simulink model "ps_model"  (R2025b)
settings: Solver=ode23tb  StartTime=0.0  StopTime=simlength  FixedStep=tc  MaxStep=tc
values from neighbouring files (symbols this model uses):
  omega_grid_emulator_nom = w_grid    (= 314.159265359)    [grid_emulator.m]
  omega_grid_nom = w_grid    (= 314.159265359)    [grid_emulator.m]
  ugrid_factor = 1    [grid_emulator.m]
  V_phase_normalization_factor = Vgrid_phase_normalization_factor    [grid_emulator.m]
  Vdc_base = 720    [grid_emulator.m]
  vn_eta_pu = 0    [grid_emulator.m]
  vn_xi_pu = 0    [grid_emulator.m]
  vp_xi_pu = 1    [grid_emulator.m]
undefined symbols (not defined in the file or in its folder): CFi, fnom, fPWM_INV, i_nom, ki_i, ki_u, kp_i, kp_u, Ld2_trafo_out, magnitude, n10, number_of_cells, omega_nom, Q, q1Kalman, q2Kalman, q3Kalman, R_RLload, Rd2_trafo_out, rKalman, tc, time_load_step, ts_afe, ts_inv, tsample, u_nom, Vdc_nom
libraries: fl_lib x120, nesl_utility x67, ee_lib x7, cstblocks x4, moving_average_filter x4, single_phase_transformer_lib x3, lithium_ion_cell_lib x1, simulink x1, threephase_inductor_lib x1
(part 1 of 4)
settings Model: SimulationMode=accelerator  Creator=dbagn  LastModifiedBy=dbagn
settings SolverCC: NumberNewtonIterations=3.0  ZeroCrossControl=DisableAll  AlgebraicLoopSolver=TrustRegion  SolverResetMethod=Robust
settings DataIOCC: SaveOutput=off  SignalLogging=off  DSMLogging=off  SaveTime=off  ReturnWorkspaceOutputs=off
settings OptimizationCC: ReuseModelBlockBuffer=off
settings DebuggingCC: UnconnectedInputMsg=warning  UnconnectedOutputMsg=warning  UnconnectedLineMsg=warning
settings ModelReferenceCC: EnableRefExpFcnMdlSchedulingChecks=on
settings SFSimCC: SimUserIncludeDirs=include  SimAnalyzeCustomCode=on
settings SFSimCC: SimCustomHeaderCode=|
  | #include "mavgflt.h"
  | #include "bemf_obsv.h"
  | #include "dqvector_pi.h"
  | #include "dqvector_pi_simulink.h"
  | #include "mavgflt_simulink.h"
  | #include "sv_pwm.h"
  | #include "bemf_obsv_simulink.h"
  | #include "bemf_obsv_load_est.h"
  | #include "bemf_obsv_load_est_simulink.h"
  | #include "sv_pwm_simulink.h"
  | #include "fb_state_machine.h"
  | #include "fb_state_machine_simulink.h"
settings SFSimCC: SimUserSources=|
  | dqvector_pi.c
  | dqvector_pi_simulink.c
  | mavgflt_simulink.c
  | mavgflt.c
  | bemf_obsv_simulink.c
  | bemf_obsv.c
  | bemf_obsv_load_est_simulink.c
  | bemf_obsv_load_est.c
  | sv_pwm.c
  | sv_pwm_simulink.c
  | fb_state_machine.c
  | fb_state_machine_simulink.c
settings RTWCC: GPUComputeCapability=3.5  DLArmComputeVersion=19.05

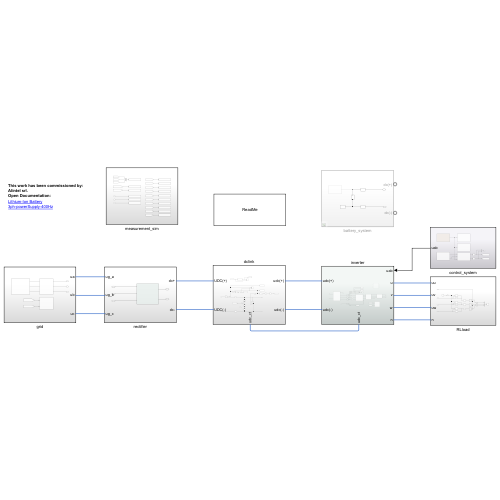
[thumbnail: Simulink's stored preview of the top-level diagram]
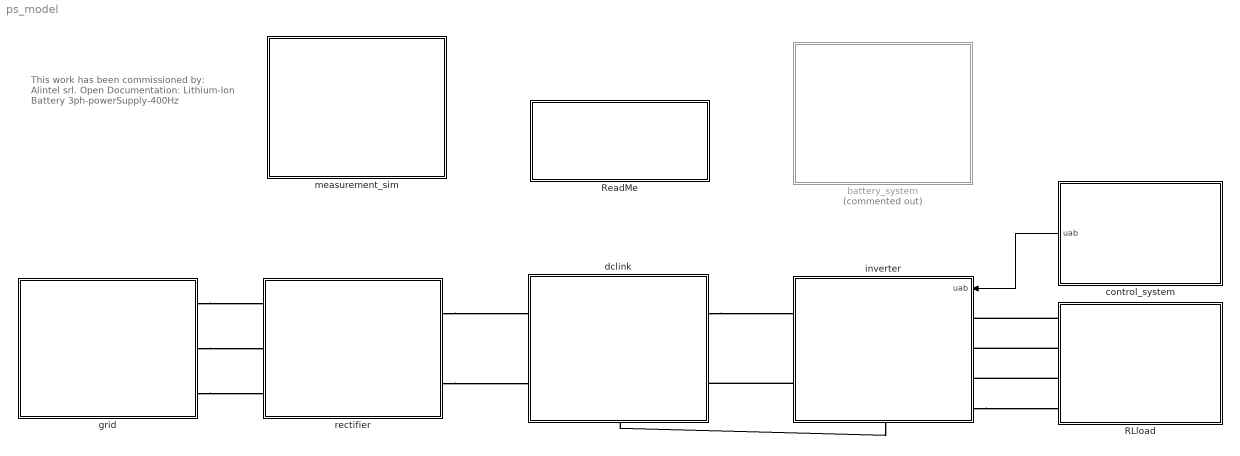
== system ps_model ==
  note: This work has been commissioned by:
      | Alintel srl.
      | Open Documentation:
      | Lithium-Ion Battery
      | 3ph-powerSupply-400Hz
  RLload : Subsystem
  ReadMe : Subsystem
      mask Display: disp('ReadMe')
  battery_system : Subsystem  Commented=on
  control_system : Subsystem
  dclink : Subsystem
      settings: PortSchema="{\"entries\":[{\"content\":{\"sides\":[{\"content\":{\"connectorIds\":[\"LConn1\",\"LConn2\"]},\"type\":\"ConnectorPlacement.EquallySpacedRectSide\",\"uuid\":\"065d3cf8-4b88-4bd8-afed-5c791b4c8227\"},{\"content\":{\"connectorIds\":[\"RConn1\",\"RConn2\"],\"side\":\"RIGHT\"},\"type\":\"ConnectorPlacement.EquallySpacedRectSide\",\"uuid\":\"93da4eee-d833-4749-b194-724bf2a8184c\"},{\"content\":{\"side\":\"TOP\"},\"type\":\"ConnectorPlacement.EquallySpacedRectSide\",\"uuid\":\"7e72ab0b-6fa9-40de-a645-1ec9cfd9e31f\"},{\"content\":{\"connectorIds\":[\"RConn3\"],\"side\":\"BOTTOM\"},\"type\":\"ConnectorPlacement.EquallySpacedRectSide\",\"uuid\":\"310375c4-299b-412a-a0fa-962bdc2b4f11\"}]},\"type\":\"ConnectorPlacement.EquallySpacedConnector\",\"uuid\":\"547429aa-4b93-405e-bc45-7aab171afd7d\"}],\"packageUris\":[\"http://schema.mathworks.com/mf0/Connector/R2020b\"],\"version\":\"1.0\"}"
  grid : Subsystem
  inverter : Subsystem
      settings: PortSchema="{\"entries\":[{\"content\":{\"sides\":[{\"content\":{\"connectorIds\":[\"In1\",\"LConn1\",\"LConn2\",\"LConn3\",\"LConn4\"]},\"type\":\"ConnectorPlacement.EquallySpacedRectSide\",\"uuid\":\"f55c1ca8-6919-4d30-91be-29ab6e5a5b93\"},{\"content\":{\"connectorIds\":[\"RConn1\",\"RConn2\"],\"side\":\"RIGHT\"},\"type\":\"ConnectorPlacement.EquallySpacedRectSide\",\"uuid\":\"500f40ac-770d-4aaa-b814-72c952c48909\"},{\"content\":{\"side\":\"TOP\"},\"type\":\"ConnectorPlacement.EquallySpacedRectSide\",\"uuid\":\"36360c7a-d142-42b5-a71d-dca271faa73f\"},{\"content\":{\"connectorIds\":[\"RConn3\"],\"side\":\"BOTTOM\"},\"type\":\"ConnectorPlacement.EquallySpacedRectSide\",\"uuid\":\"19fec778-0473-49a4-aa84-7932c0a6b289\"}]},\"type\":\"ConnectorPlacement.EquallySpacedConnector\",\"uuid\":\"7d88957d-a3a4-4eee-9ba8-53fe19feea5c\"}],\"packageUris\":[\"http://schema.mathworks.com/mf0/Connector/R2020b\"],\"version\":\"1.0\"}"
  measurement_sim : Subsystem
  rectifier : Subsystem
  wires:
  control_system/1(uab) -> inverter/1(uab)
  connections:
  rectifier/RConn1 -- dclink/LConn1
  rectifier/RConn2 -- dclink/LConn2
  inverter/RConn2 -- dclink/RConn2
  dclink/RConn1 -- inverter/RConn1
  RLload/LConn3 -- inverter/LConn3
  RLload/LConn2 -- inverter/LConn2
  RLload/LConn1 -- inverter/LConn1
  grid/RConn1 -- rectifier/LConn1
  grid/RConn2 -- rectifier/LConn2
  grid/RConn3 -- rectifier/LConn3
  inverter/RConn3 -- dclink/RConn3
  inverter/LConn4 -- RLload/LConn4

== system ps_model/RLload ==
  Bus Creator1 : BusCreator  Inputs=3
  Current Sensor : fl_lib/Electrical/Electrical Sensors/Current Sensor
  Current Sensor1 : fl_lib/Electrical/Electrical Sensors/Current Sensor
  Current Sensor2 : fl_lib/Electrical/Electrical Sensors/Current Sensor
  Inductor : ee_lib/Passive/Inductor  l=L_RLload H  enable_L_tol=0  L_tol=20  tol_distribution=1  nSigma=4  r=0 Ohm  g=1e-9 1/Ohm  enable_operating_limits=0  operating_limit_action=2  max_working_current=1 A  power_rating=1 W  i_L_specify=off  i_L_priority=High  i_L=0 A  i_L_nominal_specify=off  i_L_nominal_value=1  i_L_nominal_unit=A
  Inductor1 : ee_lib/Passive/Inductor  l=L_RLload H  enable_L_tol=0  L_tol=20  tol_distribution=1  nSigma=4  r=0 Ohm  g=1e-9 1/Ohm  enable_operating_limits=0  operating_limit_action=2  max_working_current=1 A  power_rating=1 W  i_L_specify=off  i_L_priority=High  i_L=0 A  i_L_nominal_specify=off  i_L_nominal_value=1  i_L_nominal_unit=A
  Inductor2 : ee_lib/Passive/Inductor  l=L_RLload H  enable_L_tol=0  L_tol=20  tol_distribution=1  nSigma=4  r=0 Ohm  g=1e-9 1/Ohm  enable_operating_limits=0  operating_limit_action=2  max_working_current=1 A  power_rating=1 W  i_L_specify=off  i_L_priority=High  i_L=0 A  i_L_nominal_specify=off  i_L_nominal_value=1  i_L_nominal_unit=A
  PS-Simulink Converter1 : nesl_utility/PS-Simulink Converter  PhysicalDomain=network_engine_domain  SubClassName=ps_output  LeftPortType=input  RightPortType=output  PseudoPeriodic=off  Frequencies=[]  VectorFormat=1-D array  Unit=A  AffineConversion=off
  PS-Simulink Converter2 : nesl_utility/PS-Simulink Converter  PhysicalDomain=network_engine_domain  SubClassName=ps_output  LeftPortType=input  RightPortType=output  PseudoPeriodic=off  Frequencies=[]  VectorFormat=1-D array  Unit=A  AffineConversion=off
  PS-Simulink Converter3 : nesl_utility/PS-Simulink Converter  PhysicalDomain=network_engine_domain  SubClassName=ps_output  LeftPortType=input  RightPortType=output  PseudoPeriodic=off  Frequencies=[]  VectorFormat=1-D array  Unit=A  AffineConversion=off
  Resistor : fl_lib/Electrical/Electrical Elements/Resistor  R=R_RLload Ohm  i_specify=off  i_priority=None  i=0 A  i_nominal_specify=off  i_nominal_value=1  i_nominal_unit=A  v_specify=off  v_priority=None  v=0 V  v_nominal_specify=off  v_nominal_value=1  v_nominal_unit=V
  Resistor1 : fl_lib/Electrical/Electrical Elements/Resistor  R=R_RLload Ohm  i_specify=off  i_priority=None  i=0 A  i_nominal_specify=off  i_nominal_value=1  i_nominal_unit=A  v_specify=off  v_priority=None  v=0 V  v_nominal_specify=off  v_nominal_value=1  v_nominal_unit=V
  Resistor2 : fl_lib/Electrical/Electrical Elements/Resistor  R=R_RLload Ohm  i_specify=off  i_priority=None  i=0 A  i_nominal_specify=off  i_nominal_value=1  i_nominal_unit=A  v_specify=off  v_priority=None  v=0 V  v_nominal_specify=off  v_nominal_value=1  v_nominal_unit=V
  Simulink-PS Converter : nesl_utility/Simulink-PS Converter  PhysicalDomain=network_engine_domain  SubClassName=ps_input  LeftPortType=input  RightPortType=output  PseudoPeriodic=off  Frequencies=[]  NoiseDistribution=none  NoiseParameters=[]  Unit=1  AffineConversion=off  FilteringAndDerivatives=provide  SimscapeFilterOrder=1  InputFilterTimeConstant=0.001  UdotUserProvided=0
  Step : Step  Time=time_load_step  SampleTime=0
  Switch : fl_lib/Electrical/Electrical Elements/Switch  R_closed=0.8 Ohm  G_open=1e-8 1/Ohm  Threshold=0.5  i_specify=off  i_priority=None  i=0 A  i_nominal_specify=off  i_nominal_value=1  i_nominal_unit=A  v_specify=off  v_priority=None  v=0 V  v_nominal_specify=off  v_nominal_value=1  v_nominal_unit=V
  Switch1 : fl_lib/Electrical/Electrical Elements/Switch  R_closed=0.8 Ohm  G_open=1e-8 1/Ohm  Threshold=0.5  i_specify=off  i_priority=None  i=0 A  i_nominal_specify=off  i_nominal_value=1  i_nominal_unit=A  v_specify=off  v_priority=None  v=0 V  v_nominal_specify=off  v_nominal_value=1  v_nominal_unit=V
  Switch2 : fl_lib/Electrical/Electrical Elements/Switch  R_closed=0.8 Ohm  G_open=1e-8 1/Ohm  Threshold=0.5  i_specify=off  i_priority=None  i=0 A  i_nominal_specify=off  i_nominal_value=1  i_nominal_unit=A  v_specify=off  v_priority=None  v=0 V  v_nominal_specify=off  v_nominal_value=1  v_nominal_unit=V
  iuvw_load : Scope
      settings: SampleTime=tc  ActiveDisplayYMinimum=-395.78182  ActiveDisplayYMaximum=375.94765
  uu : PMIOPort  Side=Left
  uv : PMIOPort  Port=2  Side=Left
  uw : PMIOPort  Port=3  Side=Left
  n : PMIOPort  Port=4  Side=Left
  wires:
  PS-Simulink Converter1/1 -> Bus Creator1/1  "iu_load_sim"
  Bus Creator1/1 -> iuvw_load/1
  PS-Simulink Converter3/1 -> Bus Creator1/3  "iw_load_sim"
  PS-Simulink Converter2/1 -> Bus Creator1/2  "iv_load_sim"
  Step/1 -> Simulink-PS Converter/1
  connections:
  uv/RConn1 -- Switch1/RConn2 -- Resistor1/LConn1
  Resistor/LConn1 -- uu/RConn1 -- Switch/RConn2
  uw/RConn1 -- Switch2/RConn2 -- Resistor2/LConn1
  Resistor1/RConn1 -- Switch1/LConn1 -- Inductor1/LConn1
  Switch/LConn1 -- Resistor/RConn1 -- Inductor/LConn1
  Inductor2/LConn1 -- Switch2/LConn1 -- Resistor2/RConn1
  PS-Simulink Converter3/LConn1 -- Current Sensor2/RConn1
  Current Sensor1/RConn1 -- PS-Simulink Converter2/LConn1
  Current Sensor/RConn2 -- Current Sensor2/RConn2 -- Current Sensor1/RConn2 -- n/RConn1
  Current Sensor/RConn1 -- PS-Simulink Converter1/LConn1
  Current Sensor/LConn1 -- Inductor/RConn1
  Inductor2/RConn1 -- Current Sensor2/LConn1
  Inductor1/RConn1 -- Current Sensor1/LConn1
  Switch/RConn1 -- Simulink-PS Converter/RConn1 -- Switch2/RConn1 -- Switch1/RConn1

== system ps_model/ReadMe ==

== system ps_model/battery_system ==
  DC Voltage Source : fl_lib/Electrical/Electrical Sources/DC Voltage Source  v0=Vdc_ref V
  Inductor : fl_lib/Electrical/Electrical Elements/Inductor  l=100e-6 H  r=0.025 Ohm  g=1e-9 1/Ohm  i_specify=off  i_priority=None  i=0 A  i_nominal_specify=off  i_nominal_value=1  i_nominal_unit=A  v_specify=off  v_priority=None  v=0 V  v_nominal_specify=off  v_nominal_value=1  v_nominal_unit=V  i_L_specify=off  i_L_priority=High  i_L=0 A  i_L_nominal_specify=off  i_L_nominal_value=1  i_L_nominal_unit=A
  Inductor1 : fl_lib/Electrical/Electrical Elements/Inductor  l=100e-6 H  r=0.025 Ohm  g=1e-9 1/Ohm  i_specify=off  i_priority=None  i=0 A  i_nominal_specify=off  i_nominal_value=1  i_nominal_unit=A  v_specify=off  v_priority=None  v=0 V  v_nominal_specify=off  v_nominal_value=1  v_nominal_unit=V  i_L_specify=off  i_L_priority=High  i_L=0 A  i_L_nominal_specify=off  i_L_nominal_value=1  i_L_nominal_unit=A
  Solver Configuration : nesl_utility/Solver Configuration  PhysicalDomain=network_engine_domain  SubClassName=solver  LeftPortType=input  RightPortType=generic  Tones=[]  Harmonics=[]  SimulateNoise=off  Profile=off  UseLocalSampling=off  EnableSwitchedLinearOptims=on  FrequencyDomain=off  UseCCode=off  RelTol=0.001  AbsTol=0.001  MinStep=1e-09  ToWorkspace=off  RevertToSquareIcSolve=off  NumHomotopyIterations=100  PhasorMode=off  PhasorModeNumHarmonics=1  ConsistencySolver=NEWTON_FTOL  IndexReductionMethod=DerivativeReplacement  DoDC=off  ResidualTolerance=1e-09  ConsistencyTolSource=GLOBAL  ConsistencyAbsTol=0.001  ConsistencyRelTol=0.001  ConsistencyTolFactor=0.001  UseLocalSolver=on  LocalSolverChoice=NE_BACKWARD_EULER_ADVANCER  ResolveIndetEquations=on  FunctionEvalNumThread=1  LocalSolverSampleTime=tc  DoFixedCost=on  MaxNonlinIter=5  MaxModeIter=2  ComputeImpulses=off  ImpulseIterations=2  LinearAlgebra=auto  LinearAlgebraNumThread=0  EquationFormulation=NE_TIME_EF  DelaysMemoryBudget=1024  AutomaticFiltering=on  FilteringTimeConstant=0.001  PartitionStorageMethod=AS_NEEDED  PartitionMemoryBudget=1024  PartitionMethod=ROBUST  MultibodyUseLocalSolver=off  MultibodyLocalSolverChoice=ODE1  MultibodyLocalSolverSampleTime=0.001
  battery_system : Subsystem  Commented=on
  dc(+) : PMIOPort  Side=Right
  dc(-) : PMIOPort  Port=2  Side=Right
  connections:
  Solver Configuration/RConn1 -- Inductor1/LConn1 -- DC Voltage Source/RConn1
  DC Voltage Source/LConn1 -- Inductor/LConn1 -- battery_system/RConn1
  Inductor/RConn1 -- dc(+)/RConn1
  Inductor1/RConn1 -- dc(-)/RConn1

== system ps_model/control_system ==
  Bus Creator1 : BusCreator  Inputs=2
  Unit Delay1 : UnitDelay  SampleTime=ts_inv  HasFrameUpgradeWarning=on
  Unit Delay2 : UnitDelay  SampleTime=ts_inv  HasFrameUpgradeWarning=on
  current_measure : Subsystem
  dq2alphabeta : MATLAB Function  TreatAsAtomicUnit=on  SystemSampleTime=ts_inv
  phase_gen : Subsystem
  scalar_voltage_control : Subsystem
  voltage_measure : Subsystem
  uab : Outport  VectorParamsAs1DForOutWhenUnconnected=off
  tag scope: u_alpha_ctrl_out=global, u_beta_ctrl_out=global
  wires:
  Unit Delay1/1 -> [u_alpha_ctrl_out], Bus Creator1/1  "ua"
  phase_gen/1(electrical_phase) -> current_measure/1(phase), voltage_measure/1(phase), dq2alphabeta/3(phase)
  Unit Delay2/1 -> [u_beta_ctrl_out], Bus Creator1/2  "ub"
  dq2alphabeta/1(alpha) -> Unit Delay1/1  "ua"
  Bus Creator1/1 -> uab/1
  dq2alphabeta/2(beta) -> Unit Delay2/1  "ub"
  scalar_voltage_control/1(d) -> dq2alphabeta/1(d)
  scalar_voltage_control/2(q) -> dq2alphabeta/2(q)

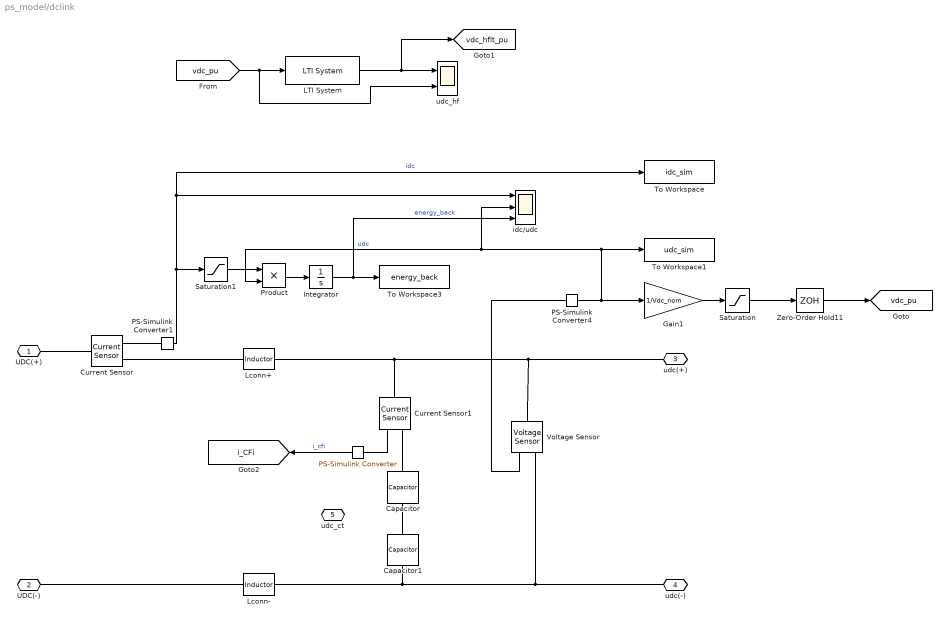
== system ps_model/dclink ==
  " " : nesl_utility/PS-Simulink Converter  PhysicalDomain=network_engine_domain  SubClassName=ps_output  LeftPortType=input  RightPortType=output  PseudoPeriodic=off  Frequencies=[]  VectorFormat=1-D array  Unit=A  AffineConversion=off
  Capacitor : fl_lib/Electrical/Electrical Elements/Capacitor  c=2*CFi F  r=1e-3 Ohm  g=0 1/Ohm  i_specify=off  i_priority=None  i=0 A  i_nominal_specify=off  i_nominal_value=1  i_nominal_unit=A  v_specify=off  v_priority=None  v=0 V  v_nominal_specify=off  v_nominal_value=1  v_nominal_unit=V  vc_specify=off  vc_priority=High  vc=0 V  vc_nominal_specify=off  vc_nominal_value=1  vc_nominal_unit=V
  Capacitor1 : fl_lib/Electrical/Electrical Elements/Capacitor  c=2*CFi F  r=1e-3 Ohm  g=0 1/Ohm  i_specify=off  i_priority=None  i=0 A  i_nominal_specify=off  i_nominal_value=1  i_nominal_unit=A  v_specify=off  v_priority=None  v=0 V  v_nominal_specify=off  v_nominal_value=1  v_nominal_unit=V  vc_specify=off  vc_priority=High  vc=0 V  vc_nominal_specify=off  vc_nominal_value=1  vc_nominal_unit=V
  Current Sensor : fl_lib/Electrical/Electrical Sensors/Current Sensor
  Current Sensor1 : fl_lib/Electrical/Electrical Sensors/Current Sensor
  Gain1 : Gain  Gain=1/Vdc_nom
  Integrator : Integrator
  LTI System : cstblocks/LTI System  sys=hpf2q_d  IC=[]  PadeOrder=0
  Lconn+ : fl_lib/Electrical/Electrical Elements/Inductor  l=0.5e-6 H  r=5e-3 Ohm  g=1e-9 1/Ohm  i_specify=on  i_priority=High  i=0 A  i_nominal_specify=off  i_nominal_value=1  i_nominal_unit=A  v_specify=off  v_priority=None  v=0 V  v_nominal_specify=off  v_nominal_value=1  v_nominal_unit=V  i_L_specify=off  i_L_priority=High  i_L=0 A  i_L_nominal_specify=off  i_L_nominal_value=1  i_L_nominal_unit=A
  Lconn- : fl_lib/Electrical/Electrical Elements/Inductor  l=0.5e-6 H  r=5e-3 Ohm  g=1e-9 1/Ohm  i_specify=on  i_priority=High  i=0 A  i_nominal_specify=off  i_nominal_value=1  i_nominal_unit=A  v_specify=off  v_priority=None  v=0 V  v_nominal_specify=off  v_nominal_value=1  v_nominal_unit=V  i_L_specify=off  i_L_priority=High  i_L=0 A  i_L_nominal_specify=off  i_L_nominal_value=1  i_L_nominal_unit=A
  PS-Simulink Converter1 : nesl_utility/PS-Simulink Converter  PhysicalDomain=network_engine_domain  SubClassName=ps_output  LeftPortType=input  RightPortType=output  PseudoPeriodic=off  Frequencies=[]  VectorFormat=1-D array  Unit=A  AffineConversion=on
  PS-Simulink Converter4 : nesl_utility/PS-Simulink Converter  PhysicalDomain=network_engine_domain  SubClassName=ps_output  LeftPortType=input  RightPortType=output  PseudoPeriodic=off  Frequencies=[]  VectorFormat=1-D array  Unit=V  AffineConversion=on
  Product : Product
  Saturation : Saturate  UpperLimit=inf  LowerLimit=0.1
  Saturation1 : Saturate  UpperLimit=0  LowerLimit=-inf
  To Workspace : ToWorkspace  VariableName=idc_sim  SampleTime=tc
      settings: MaxDataPoints=Nc
  To Workspace1 : ToWorkspace  VariableName=udc_sim  SampleTime=tc
      settings: MaxDataPoints=Nc
  To Workspace3 : ToWorkspace  VariableName=energy_back  SampleTime=tc
      settings: MaxDataPoints=Nc
  Voltage Sensor : fl_lib/Electrical/Electrical Sensors/Voltage Sensor
  Zero-Order Hold11 : ZeroOrderHold  SampleTime=ts_inv
  idc/udc : Scope  NumInputPorts=3
      settings: SampleTime=tc  ActiveDisplayYMinimum=-308.72111  ActiveDisplayYMaximum=2778.48988
  udc_hf : Scope  NumInputPorts=2
      settings: SampleTime=ts_inv  ActiveDisplayYMinimum=-0.19183  ActiveDisplayYMaximum=1.2776
  UDC(+) : PMIOPort  Side=Left
  UDC(-) : PMIOPort  Port=2  Side=Left
  udc(+) : PMIOPort  Port=3  Side=Right
  udc(-) : PMIOPort  Port=4  Side=Right
  udc_ct : PMIOPort  Port=5  Side=Right
  tag scope: i_CFi=global, vdc_hflt_pu=global, vdc_pu=global
  wires:
  Saturation/1 -> Zero-Order Hold11/1
  PS-Simulink Converter4/1 -> idc/udc/2, Product/2, To Workspace1/1, Gain1/1  "udc"
  Gain1/1 -> Saturation/1
  PS-Simulink Converter1/1 -> Saturation1/1, To Workspace/1, idc/udc/1  "idc"
  Saturation1/1 -> Product/1
  Product/1 -> Integrator/1
  Integrator/1 -> idc/udc/3, To Workspace3/1  "energy_back"
  LTI System/1 -> [vdc_hflt_pu], udc_hf/1
  [vdc_pu] -> udc_hf/2, LTI System/1
  Zero-Order Hold11/1 -> [vdc_pu]
  " "/1 -> [i_CFi]  "i_cfi"
  connections:
  PS-Simulink Converter4/LConn1 -- Voltage Sensor/RConn1
  PS-Simulink Converter1/LConn1 -- Current Sensor/RConn1
  Current Sensor/RConn2 -- Lconn+/LConn1
  Current Sensor/LConn1 -- UDC(+)/RConn1
  Lconn-/RConn1 -- UDC(-)/RConn1
  Lconn+/RConn1 -- Current Sensor1/LConn1 -- Voltage Sensor/LConn1 -- udc(+)/RConn1
  Voltage Sensor/RConn2 -- udc(-)/RConn1 -- Capacitor1/RConn1 -- Lconn-/LConn1
  Capacitor1/LConn1 -- Capacitor/RConn1
  Current Sensor1/RConn1 -- " "/LConn1
  Current Sensor1/RConn2 -- Capacitor/LConn1

== system ps_model/grid ==
  grid_emulator : Subsystem
  instantaneus_power : Subsystem
  threephase_vi_measures : Subsystem
  ua : PMIOPort  Side=Right
  ub : PMIOPort  Port=2  Side=Right
  uc : PMIOPort  Port=3  Side=Right
  wires:
  [vgrid_abc] -> instantaneus_power/1(Vline)
  [igrid_abc] -> instantaneus_power/2(Iline)
  connections:
  threephase_vi_measures/LConn3 -- grid_emulator/RConn3
  threephase_vi_measures/LConn1 -- grid_emulator/RConn1
  threephase_vi_measures/RConn2 -- ub/RConn1
  threephase_vi_measures/LConn2 -- grid_emulator/RConn2
  threephase_vi_measures/RConn1 -- ua/RConn1
  threephase_vi_measures/RConn3 -- uc/RConn1

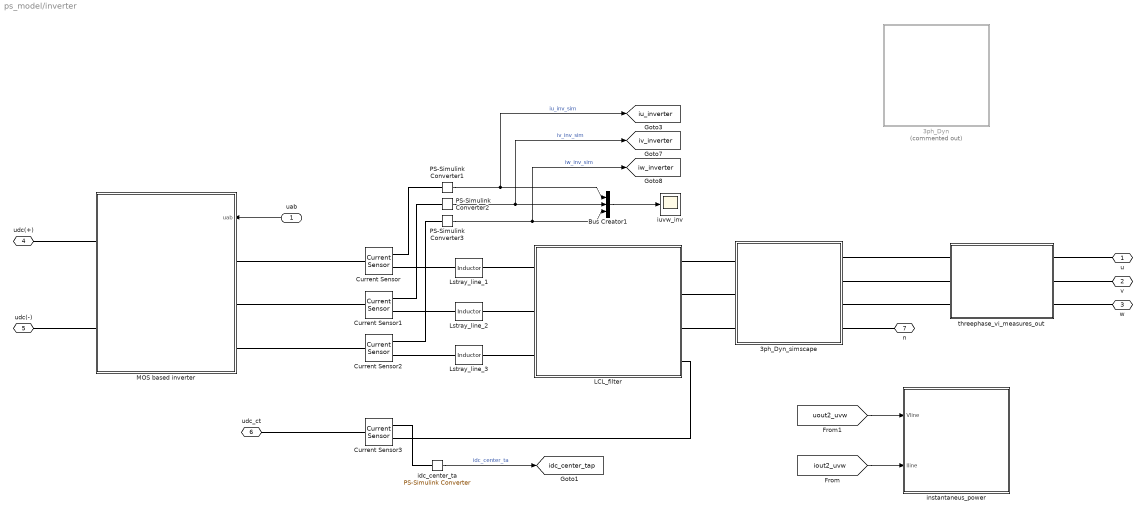
== system ps_model/inverter ==
  uab : Inport
  3ph_Dyn : Subsystem  Commented=on
  3ph_Dyn_simscape : Subsystem
  Bus Creator1 : BusCreator  Inputs=3
  Current Sensor{,1..3} (4 alike) : fl_lib/Electrical/Electrical Sensors/Current Sensor
  LCL_filter : Subsystem
  Lstray_line_1 : ee_lib/Passive/Inductor  l=5e-6 H  enable_L_tol=ee.enum.toleranceApplication.none  L_tol=20  tol_distribution=ee.enum.toleranceDistribution.uniform  nSigma=4  r=0 Ohm  g=1e-9 1/Ohm  enable_operating_limits=ee.enum.enable.no  operating_limit_action=ee.enum.passive.reportOpLim.warn  max_working_current=1 A  power_rating=1 W  i_L_specify=on  i_L_priority=High  i_L=0 A  i_L_nominal_specify=off  i_L_nominal_value=1  i_L_nominal_unit=A
  Lstray_line_2 : ee_lib/Passive/Inductor  l=5e-6 H  enable_L_tol=ee.enum.toleranceApplication.none  L_tol=20  tol_distribution=ee.enum.toleranceDistribution.uniform  nSigma=4  r=0 Ohm  g=1e-9 1/Ohm  enable_operating_limits=ee.enum.enable.no  operating_limit_action=ee.enum.passive.reportOpLim.warn  max_working_current=1 A  power_rating=1 W  i_L_specify=on  i_L_priority=High  i_L=0 A  i_L_nominal_specify=off  i_L_nominal_value=1  i_L_nominal_unit=A
  Lstray_line_3 : ee_lib/Passive/Inductor  l=5e-6 H  enable_L_tol=ee.enum.toleranceApplication.none  L_tol=20  tol_distribution=ee.enum.toleranceDistribution.uniform  nSigma=4  r=0 Ohm  g=1e-9 1/Ohm  enable_operating_limits=ee.enum.enable.no  operating_limit_action=ee.enum.passive.reportOpLim.warn  max_working_current=1 A  power_rating=1 W  i_L_specify=on  i_L_priority=High  i_L=0 A  i_L_nominal_specify=off  i_L_nominal_value=1  i_L_nominal_unit=A
  MOS based inverter : Subsystem
  PS-Simulink Converter1 : nesl_utility/PS-Simulink Converter  PhysicalDomain=network_engine_domain  SubClassName=ps_output  LeftPortType=input  RightPortType=output  PseudoPeriodic=off  Frequencies=[]  VectorFormat=1-D array  Unit=A  AffineConversion=off
  PS-Simulink Converter2 : nesl_utility/PS-Simulink Converter  PhysicalDomain=network_engine_domain  SubClassName=ps_output  LeftPortType=input  RightPortType=output  PseudoPeriodic=off  Frequencies=[]  VectorFormat=1-D array  Unit=A  AffineConversion=off
  PS-Simulink Converter3 : nesl_utility/PS-Simulink Converter  PhysicalDomain=network_engine_domain  SubClassName=ps_output  LeftPortType=input  RightPortType=output  PseudoPeriodic=off  Frequencies=[]  VectorFormat=1-D array  Unit=A  AffineConversion=off
  idc_center_ta : nesl_utility/PS-Simulink Converter  PhysicalDomain=network_engine_domain  SubClassName=ps_output  LeftPortType=input  RightPortType=output  PseudoPeriodic=off  Frequencies=[]  VectorFormat=1-D array  Unit=A  AffineConversion=off
  instantaneus_power : Subsystem
  iuvw_inv : Scope
      settings: SampleTime=tc  ActiveDisplayYMinimum=-424.46488  ActiveDisplayYMaximum=421.04569
  threephase_vi_measures_out : Subsystem
  u : PMIOPort  Side=Left
  v : PMIOPort  Port=2  Side=Left
  w : PMIOPort  Port=3  Side=Left
  udc(+) : PMIOPort  Port=4  Side=Right
  udc(-) : PMIOPort  Port=5  Side=Right
  udc_ct : PMIOPort  Port=6  Side=Right
  n : PMIOPort  Port=7  Side=Left
  tag scope: idc_center_tap=global, iu_inverter=global, iv_inverter=global, iw_inverter=global
  wires:
  Bus Creator1/1 -> iuvw_inv/1
  PS-Simulink Converter3/1 -> Bus Creator1/3, [iw_inverter]  "iw_inv_sim"
  PS-Simulink Converter1/1 -> [iu_inverter], Bus Creator1/1  "iu_inv_sim"
  PS-Simulink Converter2/1 -> [iv_inverter], Bus Creator1/2  "iv_inv_sim"
  uab/1 -> MOS based inverter/1(uab)
  idc_center_ta/1 -> [idc_center_tap]  "idc_center_ta"
  [iout2_uvw] -> instantaneus_power/2(Iline)
  [uout2_uvw] -> instantaneus_power/1(Vline)
  connections:
  Current Sensor1/LConn1 -- MOS based inverter/LConn2
  Current Sensor/LConn1 -- MOS based inverter/LConn1
  Current Sensor2/LConn1 -- MOS based inverter/LConn3
  udc(+)/RConn1 -- MOS based inverter/RConn1
  udc(-)/RConn1 -- MOS based inverter/RConn2
  PS-Simulink Converter3/LConn1 -- Current Sensor2/RConn1
  Current Sensor1/RConn1 -- PS-Simulink Converter2/LConn1
  Current Sensor1/RConn2 -- Lstray_line_2/LConn1
  Current Sensor/RConn1 -- PS-Simulink Converter1/LConn1
  Current Sensor/RConn2 -- Lstray_line_1/LConn1
  Current Sensor2/RConn2 -- Lstray_line_3/LConn1
  LCL_filter/LConn1 -- Lstray_line_1/RConn1
  LCL_filter/LConn2 -- Lstray_line_2/RConn1
  LCL_filter/LConn3 -- Lstray_line_3/RConn1
  threephase_vi_measures_out/RConn1 -- u/RConn1
  threephase_vi_measures_out/RConn2 -- v/RConn1
  threephase_vi_measures_out/RConn3 -- w/RConn1
  Current Sensor3/RConn2 -- LCL_filter/RConn4
  Current Sensor3/RConn1 -- idc_center_ta/LConn1
  udc_ct/RConn1 -- Current Sensor3/LConn1
  3ph_Dyn_simscape/RConn1 -- threephase_vi_measures_out/LConn1
  3ph_Dyn_simscape/LConn1 -- LCL_filter/RConn1
  3ph_Dyn_simscape/RConn2 -- threephase_vi_measures_out/LConn2
  3ph_Dyn_simscape/LConn2 -- LCL_filter/RConn2
  3ph_Dyn_simscape/RConn3 -- threephase_vi_measures_out/LConn3
  3ph_Dyn_simscape/LConn3 -- LCL_filter/RConn3
  3ph_Dyn_simscape/RConn4 -- n/RConn1

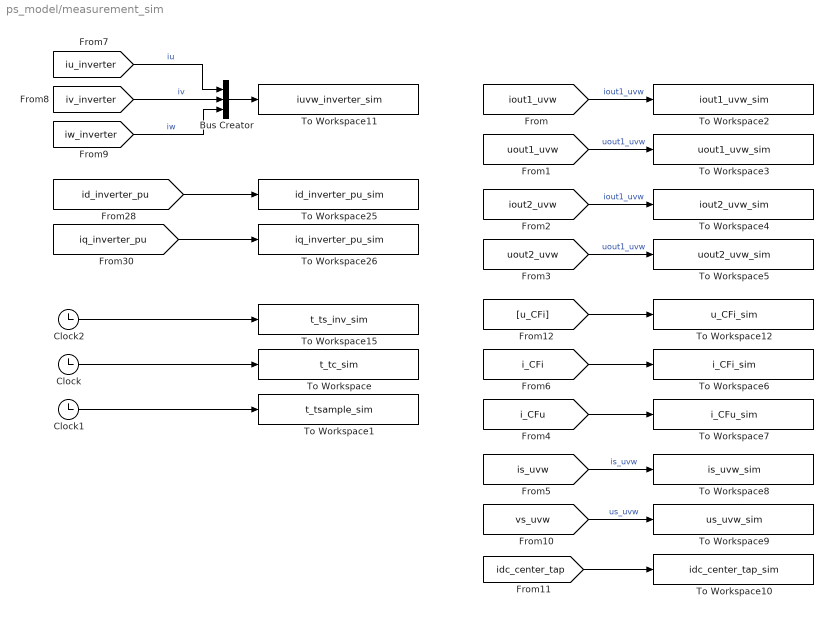
== system ps_model/measurement_sim ==
  Bus Creator : BusCreator  Inputs=3
  Clock : Clock
  Clock1 : Clock
  Clock2 : Clock
  To Workspace : ToWorkspace  VariableName=t_tc_sim  SampleTime=tc
      settings: MaxDataPoints=Nc
  To Workspace1 : ToWorkspace  VariableName=t_tsample_sim  SampleTime=tsample
      settings: MaxDataPoints=Nsample
  To Workspace10 : ToWorkspace  VariableName=idc_center_tap_sim  SampleTime=tc
      settings: MaxDataPoints=Nc
  To Workspace11 : ToWorkspace  VariableName=iuvw_inverter_sim  SampleTime=tc
      settings: MaxDataPoints=Nc
  To Workspace12 : ToWorkspace  VariableName=u_CFi_sim  SampleTime=tc
      settings: MaxDataPoints=Nc
  To Workspace15 : ToWorkspace  VariableName=t_ts_inv_sim  SampleTime=ts_inv
      settings: MaxDataPoints=Ns_inv
  To Workspace2 : ToWorkspace  VariableName=iout1_uvw_sim  SampleTime=tc
      settings: MaxDataPoints=Nc
  To Workspace25 : ToWorkspace  VariableName=id_inverter_pu_sim  SampleTime=tc
      settings: MaxDataPoints=Nc
  To Workspace26 : ToWorkspace  VariableName=iq_inverter_pu_sim  SampleTime=tc
      settings: MaxDataPoints=Nc
  To Workspace3 : ToWorkspace  VariableName=uout1_uvw_sim  SampleTime=tc
      settings: MaxDataPoints=Nc
  To Workspace4 : ToWorkspace  VariableName=iout2_uvw_sim  SampleTime=tc
      settings: MaxDataPoints=Nc
  To Workspace5 : ToWorkspace  VariableName=uout2_uvw_sim  SampleTime=tc
      settings: MaxDataPoints=Nc
  To Workspace6 : ToWorkspace  VariableName=i_CFi_sim  SampleTime=tc
      settings: MaxDataPoints=Nc
  To Workspace7 : ToWorkspace  VariableName=i_CFu_sim  SampleTime=tc
      settings: MaxDataPoints=Nc
  To Workspace8 : ToWorkspace  VariableName=is_uvw_sim  SampleTime=tc
      settings: MaxDataPoints=Nc
  To Workspace9 : ToWorkspace  VariableName=us_uvw_sim  SampleTime=tc
      settings: MaxDataPoints=Nc
  wires:
  Clock1/1 -> To Workspace1/1
  Clock/1 -> To Workspace/1
  [iv_inverter] -> Bus Creator/2  "iv"
  [iw_inverter] -> Bus Creator/3  "iw"
  [iu_inverter] -> Bus Creator/1  "iu"
  Bus Creator/1 -> To Workspace11/1
  Clock2/1 -> To Workspace15/1
  [id_inverter_pu] -> To Workspace25/1
  [iq_inverter_pu] -> To Workspace26/1
  [iout1_uvw] -> To Workspace2/1  "iout1_uvw"
  [uout1_uvw] -> To Workspace3/1  "uout1_uvw"
  [uout2_uvw] -> To Workspace5/1  "uout1_uvw"
  [iout2_uvw] -> To Workspace4/1  "iout1_uvw"
  [i_CFi] -> To Workspace6/1
  [i_CFu] -> To Workspace7/1
  [is_uvw] -> To Workspace8/1  "is_uvw"
  [vs_uvw] -> To Workspace9/1  "us_uvw"
  [idc_center_tap] -> To Workspace10/1
  [u_CFi] -> To Workspace12/1

== system ps_model/rectifier ==
  rectifier : Subsystem
  ug_a : PMIOPort  Side=Left
  dc+ : PMIOPort  Port=2  Side=Right
  ug_b : PMIOPort  Port=3  Side=Left
  dc- : PMIOPort  Port=4  Side=Right
  ug_c : PMIOPort  Port=5  Side=Left
  connections:
  dc-/RConn1 -- rectifier/RConn2
  dc+/RConn1 -- rectifier/RConn1
  rectifier/LConn1 -- ug_a/RConn1
  rectifier/LConn2 -- ug_b/RConn1
  rectifier/LConn3 -- ug_c/RConn1

== system ps_model/battery_system/battery_system ==
  Electrical Reference1 : fl_lib/Electrical/Electrical Elements/Electrical Reference
  LithiumIonBattery : Subsystem
  Uout+ : PMIOPort  Side=Right
  connections:
  LithiumIonBattery/RConn2 -- Electrical Reference1/LConn1
  LithiumIonBattery/RConn1 -- Uout+/RConn1

== system ps_model/control_system/current_measure ==
  phase : Inport
  current_transformation : Subsystem
  sample_hold_normalization : Subsystem
  wires:
  sample_hold_normalization/3(iw_pu) -> current_transformation/3(w)
  [iu_inverter] -> sample_hold_normalization/1(iu)  "iu"
  sample_hold_normalization/1(iu_pu) -> current_transformation/1(u)
  [iv_inverter] -> sample_hold_normalization/2(iv)  "iv"
  [iw_inverter] -> sample_hold_normalization/3(iw)  "iw"
  phase/1 -> current_transformation/4(phase)
  sample_hold_normalization/2(iv_pu) -> current_transformation/2(v)

== system ps_model/control_system/phase_gen ==
  Constant4 : Constant  Value=2*pi*fnom
  Sum4 : Sum  SaturateOnIntegerOverflow=on
  Unit Delay1 : UnitDelay  SampleTime=ts_inv  HasFrameUpgradeWarning=on
  bounder1 : MATLAB Function  TreatAsAtomicUnit=on  SystemSampleTime=ts_inv
  kp2 : Gain  Gain=ts_inv  SaturateOnIntegerOverflow=on  OutDataTypeStr=Inherit: Same as input  ParamDataTypeStr=Inherit: Same as input
  electrical_phase : Outport
  wires:
  Unit Delay1/1 -> Sum4/2
  Constant4/1 -> kp2/1
  kp2/1 -> Sum4/1
  bounder1/1(y) -> Unit Delay1/1, electrical_phase/1
  Sum4/1 -> bounder1/1(u)

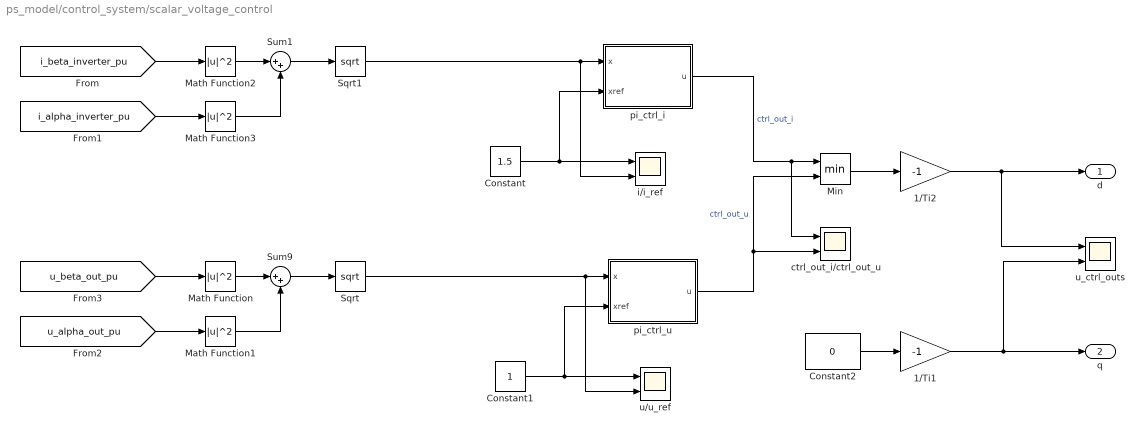
== system ps_model/control_system/scalar_voltage_control ==
  1/Ti1 : Gain  Gain=-1  SaturateOnIntegerOverflow=on  OutDataTypeStr=Inherit: Same as input  ParamDataTypeStr=Inherit: Same as input
  1/Ti2 : Gain  Gain=-1  SaturateOnIntegerOverflow=on  OutDataTypeStr=Inherit: Same as input  ParamDataTypeStr=Inherit: Same as input
  Constant : Constant  Value=1.5
  Constant1 : Constant
  Constant2 : Constant  Value=0  SampleTime=ts_inv
  Math Function{,1..3} (4 alike) : Math  Operator=magnitude^2  SignedPower=on
  Min : MinMax  Inputs=2
  Sqrt : Sqrt
  Sqrt1 : Sqrt
  Sum1 : Sum  Inputs=|++
  Sum9 : Sum  Inputs=|++
  ctrl_out_i/ctrl_out_u : Scope  NumInputPorts=2
      settings: SampleTime=tc  ActiveDisplayYMinimum=0.45437  ActiveDisplayYMaximum=1.06062
  i/i_ref : Scope  NumInputPorts=2
      settings: SampleTime=tc  ActiveDisplayYMinimum=-0.1875  ActiveDisplayYMaximum=1.6875  DataLoggingVariableName=ScopeData2
  pi_ctrl_i : Subsystem  mask{kp=kp_i, ki=ki_i, ts=ts_inv, sat_pos=1, sat_neg=0}
  pi_ctrl_u : Subsystem  mask{kp=kp_u, ki=ki_u, ts=ts_inv, sat_pos=1, sat_neg=0}
  u/u_ref : Scope  NumInputPorts=2
      settings: SampleTime=tc  ActiveDisplayYMinimum=-0.15142  ActiveDisplayYMaximum=1.3628
  u_ctrl_outs : Scope  NumInputPorts=2
      settings: SampleTime=tc  ActiveDisplayYMinimum=-0.40236  ActiveDisplayYMaximum=0.04471
  d : Outport
  q : Outport  Port=2
  wires:
  [u_alpha_out_pu] -> Math Function1/1
  Math Function/1 -> Sum9/1
  Sum9/1 -> Sqrt/1
  [u_beta_out_pu] -> Math Function/1
  Math Function1/1 -> Sum9/2
  Min/1 -> 1/Ti2/1
  1/Ti1/1 -> q/1, u_ctrl_outs/2
  Constant1/1 -> u/u_ref/1, pi_ctrl_u/2(xref)
  Sqrt/1 -> u/u_ref/2, pi_ctrl_u/1(x)
  Sqrt1/1 -> pi_ctrl_i/1(x), i/i_ref/2
  Constant/1 -> i/i_ref/1, pi_ctrl_i/2(xref)
  Math Function3/1 -> Sum1/2
  [i_beta_inverter_pu] -> Math Function2/1
  Sum1/1 -> Sqrt1/1
  Math Function2/1 -> Sum1/1
  [i_alpha_inverter_pu] -> Math Function3/1
  Constant2/1 -> 1/Ti1/1
  pi_ctrl_u/1(u) -> Min/2, ctrl_out_i/ctrl_out_u/2  "ctrl_out_u"
  pi_ctrl_i/1(u) -> ctrl_out_i/ctrl_out_u/1, Min/1  "ctrl_out_i"
  1/Ti2/1 -> u_ctrl_outs/1, d/1

== system ps_model/control_system/voltage_measure ==
  phase : Inport
  Demux : Demux  Outputs=3
  sample_hold_normalization : Subsystem
  voltage_transformation : Subsystem
  wires:
  sample_hold_normalization/2(uv_pu) -> voltage_transformation/2(v)
  phase/1 -> voltage_transformation/4(phase)
  Demux/3 -> sample_hold_normalization/3(iw)  "uout_w"
  Demux/2 -> sample_hold_normalization/2(iv)  "uout_v"
  sample_hold_normalization/1(uu_pu) -> voltage_transformation/1(u)
  Demux/1 -> sample_hold_normalization/1(iu)  "uout_u"
  sample_hold_normalization/3(uw_pu) -> voltage_transformation/3(w)
  [uout2_uvw] -> Demux/1  "uout_uvw"

== system ps_model/grid/grid_emulator ==
  Controlled Voltage Source : fl_lib/Electrical/Electrical Sources/Controlled Voltage Source
  Controlled Voltage Source1 : fl_lib/Electrical/Electrical Sources/Controlled Voltage Source
  Controlled Voltage Source2 : fl_lib/Electrical/Electrical Sources/Controlled Voltage Source
  Electrical Reference : fl_lib/Electrical/Electrical Elements/Electrical Reference
  Inductor : fl_lib/Electrical/Electrical Elements/Inductor  l=10e-6 H  r=0 Ohm  g=1e-3 1/Ohm  i_specify=off  i_priority=None  i=0 A  i_nominal_specify=off  i_nominal_value=1  i_nominal_unit=A  v_specify=off  v_priority=None  v=0 V  v_nominal_specify=off  v_nominal_value=1  v_nominal_unit=V  i_L_specify=off  i_L_priority=High  i_L=0 A  i_L_nominal_specify=off  i_L_nominal_value=1  i_L_nominal_unit=A
  Inductor1 : fl_lib/Electrical/Electrical Elements/Inductor  l=10e-6 H  r=0 Ohm  g=1e-3 1/Ohm  i_specify=off  i_priority=None  i=0 A  i_nominal_specify=off  i_nominal_value=1  i_nominal_unit=A  v_specify=off  v_priority=None  v=0 V  v_nominal_specify=off  v_nominal_value=1  v_nominal_unit=V  i_L_specify=off  i_L_priority=High  i_L=0 A  i_L_nominal_specify=off  i_L_nominal_value=1  i_L_nominal_unit=A
  Inductor2 : fl_lib/Electrical/Electrical Elements/Inductor  l=10e-6 H  r=0 Ohm  g=1e-3 1/Ohm  i_specify=off  i_priority=None  i=0 A  i_nominal_specify=off  i_nominal_value=1  i_nominal_unit=A  v_specify=off  v_priority=None  v=0 V  v_nominal_specify=off  v_nominal_value=1  v_nominal_unit=V  i_L_specify=off  i_L_priority=High  i_L=0 A  i_L_nominal_specify=off  i_L_nominal_value=1  i_L_nominal_unit=A
  Inductor3 : fl_lib/Electrical/Electrical Elements/Inductor  l=1e-6 H  r=0 Ohm  g=1e-3 1/Ohm  i_specify=off  i_priority=None  i=0 A  i_nominal_specify=off  i_nominal_value=1  i_nominal_unit=A  v_specify=off  v_priority=None  v=0 V  v_nominal_specify=off  v_nominal_value=1  v_nominal_unit=V  i_L_specify=off  i_L_priority=High  i_L=0 A  i_L_nominal_specify=off  i_L_nominal_value=1  i_L_nominal_unit=A
  Inductor4 : fl_lib/Electrical/Electrical Elements/Inductor  l=1e-6 H  r=0 Ohm  g=1e-3 1/Ohm  i_specify=off  i_priority=None  i=0 A  i_nominal_specify=off  i_nominal_value=1  i_nominal_unit=A  v_specify=off  v_priority=None  v=0 V  v_nominal_specify=off  v_nominal_value=1  v_nominal_unit=V  i_L_specify=off  i_L_priority=High  i_L=0 A  i_L_nominal_specify=off  i_L_nominal_value=1  i_L_nominal_unit=A
  Inductor5 : fl_lib/Electrical/Electrical Elements/Inductor  l=1e-6 H  r=0 Ohm  g=1e-3 1/Ohm  i_specify=off  i_priority=None  i=0 A  i_nominal_specify=off  i_nominal_value=1  i_nominal_unit=A  v_specify=off  v_priority=None  v=0 V  v_nominal_specify=off  v_nominal_value=1  v_nominal_unit=V  i_L_specify=off  i_L_priority=High  i_L=0 A  i_L_nominal_specify=off  i_L_nominal_value=1  i_L_nominal_unit=A
  Simulink-PS Converter : nesl_utility/Simulink-PS Converter  PhysicalDomain=network_engine_domain  SubClassName=ps_input  LeftPortType=input  RightPortType=output  PseudoPeriodic=off  Frequencies=[]  NoiseDistribution=none  NoiseParameters=[]  Unit=V  AffineConversion=off  FilteringAndDerivatives=provide  SimscapeFilterOrder=1  InputFilterTimeConstant=0.001  UdotUserProvided=0
  Simulink-PS Converter1 : nesl_utility/Simulink-PS Converter  PhysicalDomain=network_engine_domain  SubClassName=ps_input  LeftPortType=input  RightPortType=output  PseudoPeriodic=off  Frequencies=[]  NoiseDistribution=none  NoiseParameters=[]  Unit=V  AffineConversion=off  FilteringAndDerivatives=provide  SimscapeFilterOrder=1  InputFilterTimeConstant=0.001  UdotUserProvided=0
  Simulink-PS Converter2 : nesl_utility/Simulink-PS Converter  PhysicalDomain=network_engine_domain  SubClassName=ps_input  LeftPortType=input  RightPortType=output  PseudoPeriodic=off  Frequencies=[]  NoiseDistribution=none  NoiseParameters=[]  Unit=V  AffineConversion=off  FilteringAndDerivatives=provide  SimscapeFilterOrder=1  InputFilterTimeConstant=0.001  UdotUserProvided=0
  Solver Configuration : nesl_utility/Solver Configuration  PhysicalDomain=network_engine_domain  SubClassName=solver  LeftPortType=input  RightPortType=generic  Tones=[]  Harmonics=[]  SimulateNoise=off  Profile=off  UseLocalSampling=off  EnableSwitchedLinearOptims=on  FrequencyDomain=off  UseCCode=off  RelTol=0.001  AbsTol=0.001  MinStep=1e-09  ToWorkspace=off  RevertToSquareIcSolve=off  NumHomotopyIterations=100  PhasorMode=off  PhasorModeNumHarmonics=1  ConsistencySolver=NEWTON_XTOL_AFTER_FTOL  IndexReductionMethod=DerivativeReplacement  DoDC=on  ResidualTolerance=1e-09  ConsistencyTolSource=GLOBAL  ConsistencyAbsTol=0.001  ConsistencyRelTol=0.001  ConsistencyTolFactor=0.001  UseLocalSolver=on  LocalSolverChoice=NE_BACKWARD_EULER_ADVANCER  ResolveIndetEquations=on  FunctionEvalNumThread=1  LocalSolverSampleTime=tc  DoFixedCost=on  MaxNonlinIter=3  MaxModeIter=2  ComputeImpulses=off  ImpulseIterations=2  LinearAlgebra=auto  LinearAlgebraNumThread=0  EquationFormulation=NE_TIME_EF  DelaysMemoryBudget=1024  AutomaticFiltering=on  FilteringTimeConstant=0.001  PartitionStorageMethod=AS_NEEDED  PartitionMemoryBudget=1024  PartitionMethod=ROBUST  MultibodyUseLocalSolver=off  MultibodyLocalSolverChoice=ODE1  MultibodyLocalSolverSampleTime=0.001
  grid_emulator : Subsystem
  threephase_vi_measures_mv : Subsystem
  u1 : PMIOPort  Side=Right
  u2 : PMIOPort  Port=2  Side=Right
  u3 : PMIOPort  Port=3  Side=Right
  wires:
  grid_emulator/2(Vmb) -> Simulink-PS Converter1/1
  grid_emulator/3(Vmc) -> Simulink-PS Converter2/1
  grid_emulator/1(Vma) -> Simulink-PS Converter/1
  connections:
  Simulink-PS Converter/RConn1 -- Controlled Voltage Source/RConn1
  Simulink-PS Converter1/RConn1 -- Controlled Voltage Source1/RConn1
  Simulink-PS Converter2/RConn1 -- Controlled Voltage Source2/RConn1
  Electrical Reference/LConn1 -- Solver Configuration/RConn1 -- Controlled Voltage Source/RConn2 -- Controlled Voltage Source1/RConn2 -- Controlled Voltage Source2/RConn2
  Controlled Voltage Source/LConn1 -- Inductor/LConn1
  Inductor1/LConn1 -- Controlled Voltage Source1/LConn1
  Inductor2/LConn1 -- Controlled Voltage Source2/LConn1
  u1/RConn1 -- Inductor3/RConn1
  u2/RConn1 -- Inductor4/RConn1
  u3/RConn1 -- Inductor5/RConn1
  Inductor/RConn1 -- threephase_vi_measures_mv/LConn1
  Inductor1/RConn1 -- threephase_vi_measures_mv/LConn2
  Inductor2/RConn1 -- threephase_vi_measures_mv/LConn3
  Inductor3/LConn1 -- threephase_vi_measures_mv/RConn1
  Inductor4/LConn1 -- threephase_vi_measures_mv/RConn2
  Inductor5/LConn1 -- threephase_vi_measures_mv/RConn3

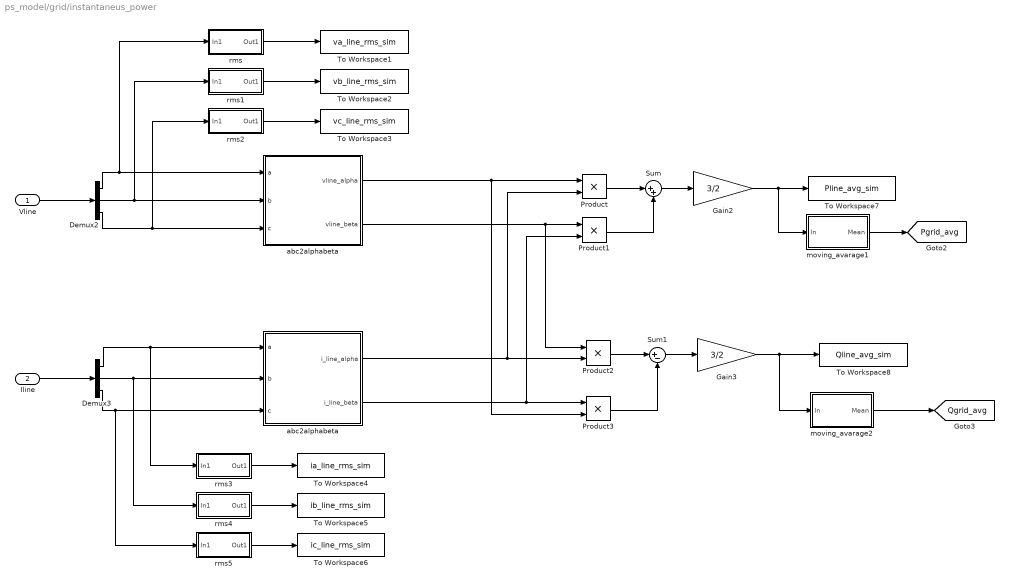
== system ps_model/grid/instantaneus_power ==
  Vline : Inport
  Iline : Inport  Port=2
  Demux2 : Demux  Outputs=3
  Demux3 : Demux  Outputs=3
  Gain2 : Gain  Gain=3/2
  Gain3 : Gain  Gain=3/2
  Product{,1..3} (4 alike) : Product  RndMeth=Zero
  Sum : Sum  Inputs=|++
  Sum1 : Sum  Inputs=|+-
  To Workspace1 : ToWorkspace  VariableName=va_line_rms_sim  SampleTime=ts_afe
      settings: MaxDataPoints=Ns_afe
  To Workspace2 : ToWorkspace  VariableName=vb_line_rms_sim  SampleTime=ts_afe
      settings: MaxDataPoints=Ns_afe
  To Workspace3 : ToWorkspace  VariableName=vc_line_rms_sim  SampleTime=ts_afe
      settings: MaxDataPoints=Ns_afe
  To Workspace4 : ToWorkspace  VariableName=ia_line_rms_sim  SampleTime=ts_afe
      settings: MaxDataPoints=Ns_afe
  To Workspace5 : ToWorkspace  VariableName=ib_line_rms_sim  SampleTime=ts_afe
      settings: MaxDataPoints=Ns_afe
  To Workspace6 : ToWorkspace  VariableName=ic_line_rms_sim  SampleTime=ts_afe
      settings: MaxDataPoints=Ns_afe
  To Workspace7 : ToWorkspace  VariableName=Pline_avg_sim  SampleTime=ts_afe
      settings: MaxDataPoints=Ns_afe
  To Workspace8 : ToWorkspace  VariableName=Qline_avg_sim  SampleTime=ts_afe
      settings: MaxDataPoints=Ns_afe
  abc2alphabeta : Subsystem
  "abc2alphabeta " : Subsystem
  moving_avarage1 : Subsystem
  moving_avarage2 : Subsystem
  rms : Subsystem
  rms1 : Subsystem
  rms2 : Subsystem
  rms3 : Subsystem
  rms4 : Subsystem
  rms5 : Subsystem
  tag scope: Pgrid_avg=global, Qgrid_avg=global
  wires:
  Gain3/1 -> moving_avarage2/1(In), To Workspace8/1
  Gain2/1 -> moving_avarage1/1(In), To Workspace7/1
  Demux2/1 -> rms/1(In1), abc2alphabeta/1(a)
  Vline/1 -> Demux2/1
  Iline/1 -> Demux3/1
  abc2alphabeta/2(vline_beta) -> Product1/1, Product2/1
  "abc2alphabeta "/2(i_line_beta) -> Product3/1, Product1/2
  abc2alphabeta/1(vline_alpha) -> Product/1, Product3/2
  "abc2alphabeta "/1(i_line_alpha) -> Product2/2, Product/2
  Product/1 -> Sum/1
  Product1/1 -> Sum/2
  Product2/1 -> Sum1/1
  Product3/1 -> Sum1/2
  Sum1/1 -> Gain3/1
  Sum/1 -> Gain2/1
  Demux2/2 -> rms1/1(In1), abc2alphabeta/2(b)
  Demux2/3 -> rms2/1(In1), abc2alphabeta/3(c)
  Demux3/1 -> "abc2alphabeta "/1(a), rms3/1(In1)
  Demux3/2 -> "abc2alphabeta "/2(b), rms4/1(In1)
  Demux3/3 -> rms5/1(In1), "abc2alphabeta "/3(c)
  moving_avarage1/1(Mean) -> [Pgrid_avg]
  moving_avarage2/1(Mean) -> [Qgrid_avg]
  rms/1(Out1) -> To Workspace1/1
  rms2/1(Out1) -> To Workspace3/1
  rms1/1(Out1) -> To Workspace2/1
  rms5/1(Out1) -> To Workspace6/1
  rms4/1(Out1) -> To Workspace5/1
  rms3/1(Out1) -> To Workspace4/1

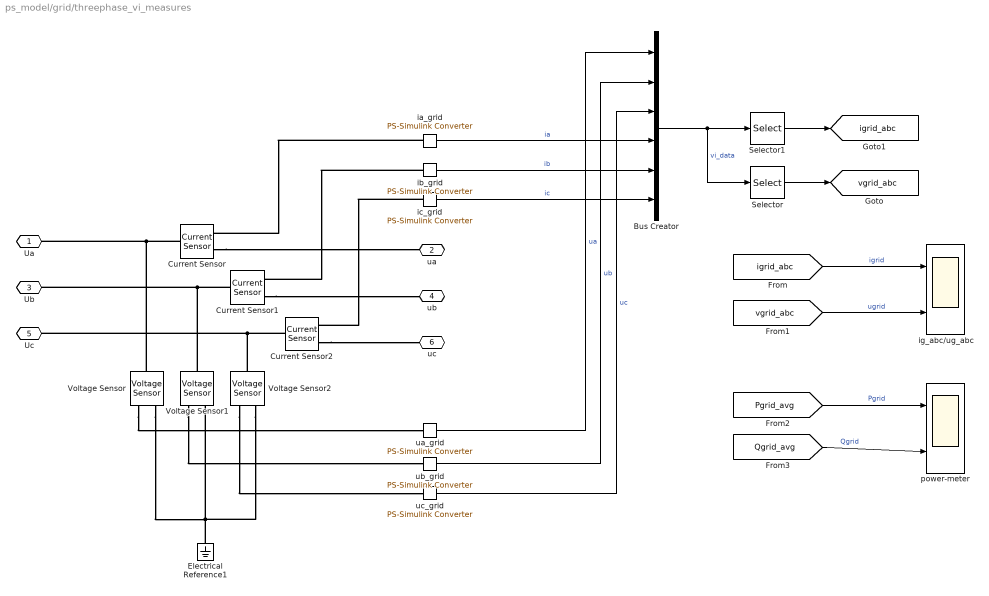
== system ps_model/grid/threephase_vi_measures ==
  Bus Creator : BusCreator  Inputs=6
  Current Sensor : fl_lib/Electrical/Electrical Sensors/Current Sensor
  Current Sensor1 : fl_lib/Electrical/Electrical Sensors/Current Sensor
  Current Sensor2 : fl_lib/Electrical/Electrical Sensors/Current Sensor
  Electrical Reference1 : fl_lib/Electrical/Electrical Elements/Electrical Reference
  Selector : Selector  InputPortWidth=6  IndexOptions=Index vector (dialog)  Indices=[1 2 3]  OutputSizes=1
  Selector1 : Selector  InputPortWidth=6  IndexOptions=Index vector (dialog)  Indices=[4 5 6]  OutputSizes=1
  Voltage Sensor : fl_lib/Electrical/Electrical Sensors/Voltage Sensor
  Voltage Sensor1 : fl_lib/Electrical/Electrical Sensors/Voltage Sensor
  Voltage Sensor2 : fl_lib/Electrical/Electrical Sensors/Voltage Sensor
  ia_grid : nesl_utility/PS-Simulink Converter  PhysicalDomain=network_engine_domain  SubClassName=ps_output  LeftPortType=input  RightPortType=output  PseudoPeriodic=off  Frequencies=[]  VectorFormat=1-D array  Unit=A  AffineConversion=off
  ib_grid : nesl_utility/PS-Simulink Converter  PhysicalDomain=network_engine_domain  SubClassName=ps_output  LeftPortType=input  RightPortType=output  PseudoPeriodic=off  Frequencies=[]  VectorFormat=1-D array  Unit=A  AffineConversion=off
  ic_grid : nesl_utility/PS-Simulink Converter  PhysicalDomain=network_engine_domain  SubClassName=ps_output  LeftPortType=input  RightPortType=output  PseudoPeriodic=off  Frequencies=[]  VectorFormat=1-D array  Unit=A  AffineConversion=off
  ig_abc/ug_abc : Scope  NumInputPorts=2
      settings: SampleTime=tc  ActiveDisplayYMinimum=-3087.53598  ActiveDisplayYMaximum=3087.53598  DataLoggingVariableName=ScopeData2
  power-meter : Scope  NumInputPorts=2
      settings: SampleTime=tc  ActiveDisplayYMinimum=-12243.78467  ActiveDisplayYMaximum=110194.06207  DataLoggingVariableName=ScopeData3
  ua_grid : nesl_utility/PS-Simulink Converter  PhysicalDomain=network_engine_domain  SubClassName=ps_output  LeftPortType=input  RightPortType=output  PseudoPeriodic=off  Frequencies=[]  VectorFormat=1-D array  Unit=V  AffineConversion=off
  ub_grid : nesl_utility/PS-Simulink Converter  PhysicalDomain=network_engine_domain  SubClassName=ps_output  LeftPortType=input  RightPortType=output  PseudoPeriodic=off  Frequencies=[]  VectorFormat=1-D array  Unit=V  AffineConversion=off
  uc_grid : nesl_utility/PS-Simulink Converter  PhysicalDomain=network_engine_domain  SubClassName=ps_output  LeftPortType=input  RightPortType=output  PseudoPeriodic=off  Frequencies=[]  VectorFormat=1-D array  Unit=V  AffineConversion=off
  Ua : PMIOPort  Side=Left
  ua : PMIOPort  Port=2  Side=Right
  Ub : PMIOPort  Port=3  Side=Left
  ub : PMIOPort  Port=4  Side=Right
  Uc : PMIOPort  Port=5  Side=Left
  uc : PMIOPort  Port=6  Side=Right
  tag scope: igrid_abc=global, vgrid_abc=global
  wires:
  Bus Creator/1 -> Selector1/1, Selector/1  "vi_data"
  Selector/1 -> [vgrid_abc]
  ib_grid/1 -> Bus Creator/5  "ib"
  ia_grid/1 -> Bus Creator/4  "ia"
  ic_grid/1 -> Bus Creator/6  "ic"
  ua_grid/1 -> Bus Creator/1  "ua"
  ub_grid/1 -> Bus Creator/2  "ub"
  uc_grid/1 -> Bus Creator/3  "uc"
  Selector1/1 -> [igrid_abc]
  [vgrid_abc] -> ig_abc/ug_abc/2  "ugrid"
  [igrid_abc] -> ig_abc/ug_abc/1  "igrid"
  [Pgrid_avg] -> power-meter/1  "Pgrid"
  [Qgrid_avg] -> power-meter/2  "Qgrid"
  connections:
  Current Sensor1/LConn1 -- Ub/RConn1 -- Voltage Sensor1/LConn1
  Electrical Reference1/LConn1 -- Voltage Sensor/RConn2 -- Voltage Sensor2/RConn2 -- Voltage Sensor1/RConn2
  Voltage Sensor/RConn1 -- ua_grid/LConn1
  Current Sensor/RConn2 -- ua/RConn1
  Voltage Sensor1/RConn1 -- ub_grid/LConn1
  Voltage Sensor2/LConn1 -- Current Sensor2/LConn1 -- Uc/RConn1
  Current Sensor/LConn1 -- Ua/RConn1 -- Voltage Sensor/LConn1
  Current Sensor1/RConn2 -- ub/RConn1
  Voltage Sensor2/RConn1 -- uc_grid/LConn1
  ib_grid/LConn1 -- Current Sensor1/RConn1
  ia_grid/LConn1 -- Current Sensor/RConn1
  ic_grid/LConn1 -- Current Sensor2/RConn1
  Current Sensor2/RConn2 -- uc/RConn1

== system ps_model/inverter/3ph_Dyn ==
  Electrical Reference1 : fl_lib/Electrical/Electrical Elements/Electrical Reference
  Inductor : fl_lib/Electrical/Electrical Elements/Inductor  l=Ld2_trafo_out H  r=Rd2_trafo_out Ohm  g=1e-9 1/Ohm  i_specify=on  i_priority=High  i=0 A  i_nominal_specify=off  i_nominal_value=1  i_nominal_unit=A  v_specify=off  v_priority=None  v=0 V  v_nominal_specify=off  v_nominal_value=1  v_nominal_unit=V  i_L_specify=off  i_L_priority=High  i_L=0 A  i_L_nominal_specify=off  i_L_nominal_value=1  i_L_nominal_unit=A
  Inductor1 : fl_lib/Electrical/Electrical Elements/Inductor  l=Ld2_trafo_out H  r=Rd2_trafo_out Ohm  g=1e-9 1/Ohm  i_specify=on  i_priority=High  i=0 A  i_nominal_specify=off  i_nominal_value=1  i_nominal_unit=A  v_specify=off  v_priority=None  v=0 V  v_nominal_specify=off  v_nominal_value=1  v_nominal_unit=V  i_L_specify=off  i_L_priority=High  i_L=0 A  i_L_nominal_specify=off  i_L_nominal_value=1  i_L_nominal_unit=A
  Inductor2 : fl_lib/Electrical/Electrical Elements/Inductor  l=Ld2_trafo_out H  r=Rd2_trafo_out Ohm  g=1e-9 1/Ohm  i_specify=on  i_priority=High  i=0 A  i_nominal_specify=off  i_nominal_value=1  i_nominal_unit=A  v_specify=off  v_priority=None  v=0 V  v_nominal_specify=off  v_nominal_value=1  v_nominal_unit=V  i_L_specify=off  i_L_priority=High  i_L=0 A  i_L_nominal_specify=off  i_L_nominal_value=1  i_L_nominal_unit=A
  Two-Winding Transformer (Three-Phase) : ee_lib/Passive/Transformers/Two-Winding Transformer (Three-Phase)  SRated=95e3 A*V  FRated=400 Hz  Winding1Connection=ee.enum.windingconnection.delta11  VRated1=250 V  Winding2Connection=ee.enum.windingconnection.Yn  VRated2=200 V  CoreType=ee.enum.coretype.threelimb  pu_Rw1=0.01  pu_Rw2=0.01  leakage_reactance_option=ee.enum.transformer_leakage.exclude  pu_Xl1=0.05  pu_Xl2=0.05  magnetizing_resistance_option=ee.enum.transformer_magnetizingResistance.exclude  pu_Rm=500  magnetizing_reactance_option=ee.enum.transformer_magnetizingReactance.exclude  saturation_option=ee.enum.transformer_saturation.exclude  pu_Xm=500  current_data=[0, .002, 1, 2]  magnetic_flux_data=[0, 1.2, 1.5, 1.51]  pu_X0=0.5  i1_specify=off  i1_priority=None  i1=[0, 0, 0] A  i1_nominal_specify=off  i1_nominal_value=1  i1_nominal_unit=A  i2_specify=off  i2_priority=None  i2=[0, 0, 0] A  i2_nominal_specify=off  i2_nominal_value=1  i2_nominal_unit=A  phi_specify=off  phi_priority=None  phi=[0, 0, 0]  phi_nominal_specify=off  phi_nominal_value=1  phi_nominal_unit=1  power_dissipated_specify=off  power_dissipated_priority=None  power_dissipated=0 W  power_dissipated_nominal_specify=off  power_dissipated_nominal_value=1  power_dissipated_nominal_unit=W
      settings: InternalSimscapePortConfiguration="{\"Bottom\":[],\"Left\":[{\"id\":\"a1\",\"label\":\"a1\",\"type\":\"foundation.electrical.electrical\"},{\"id\":\"b1\",\"label\":\"b1\",\"type\":\"foundation.electrical.electrical\"},{\"id\":\"c1\",\"label\":\"c1\",\"type\":\"foundation.electrical.electrical\"}],\"Right\":[{\"id\":\"a2\",\"label\":\"a2\",\"type\":\"foundation.electrical.electrical\"},{\"id\":\"b2\",\"label\":\"b2\",\"type\":\"foundation.electrical.electrical\"},{\"id\":\"c2\",\"label\":\"c2\",\"type\":\"foundation.electrical.electrical\"},{\"id\":\"n2\",\"label\":\"n2\",\"type\":\"foundation.electrical.electrical\"}],\"Top\":[]}"
  u : PMIOPort  Side=Right
  U : PMIOPort  Port=2  Side=Left
  v : PMIOPort  Port=3  Side=Right
  V : PMIOPort  Port=4  Side=Left
  w : PMIOPort  Port=5  Side=Right
  W : PMIOPort  Port=6  Side=Left
  n : PMIOPort  Port=7  Side=Right
  connections:
  Two-Winding Transformer (Three-Phase)/RConn4 -- n/RConn1 -- Electrical Reference1/LConn1
  Two-Winding Transformer (Three-Phase)/RConn1 -- Inductor/LConn1
  Inductor/RConn1 -- u/RConn1
  Inductor1/LConn1 -- Two-Winding Transformer (Three-Phase)/RConn2
  Inductor2/LConn1 -- Two-Winding Transformer (Three-Phase)/RConn3
  Two-Winding Transformer (Three-Phase)/LConn3 -- W/RConn1
  Two-Winding Transformer (Three-Phase)/LConn1 -- U/RConn1
  Inductor2/RConn1 -- w/RConn1
  Two-Winding Transformer (Three-Phase)/LConn2 -- V/RConn1
  Inductor1/RConn1 -- v/RConn1
